simulink library "Contact_Forces_Lib"  (R2025a)
settings: Solver=ode45  StartTime=0.0  StopTime=10.0  RelTol=1e-3  EnableMultiTasking=on
undefined symbols (not defined in the file or in its folder): b_contact, custom_param_1, custom_param_2, Extr_Data_Ring, k_contact, l_cone, length_cylinder, length_tube, mu_kinetic, mu_static, pen_exponent, pen_full_damp_F, rad_s_cone, radius_cylinder, radius_tube, v_thr, X, Y, Z
libraries: nesl_utility x197, sm_lib x115, $bdroot x72, simulink x20, fl_lib x4
(part 3 of 12)

== system Contact_Forces_Lib/2D/Circle to Circle Force Enabled ==
  In : Inport
  Bus Creator : BusCreator  Inputs=7
  Bus Creator1 : BusCreator  Inputs=3
  Bus Selector1 : BusSelector  OutputSignals=Enable
  Calculate Penetration : Subsystem
  External Force and Torque CirB : sm_lib/Forces and Torques/External Force and Torque  EnableForceX=on  EnableForceY=on  EnableForceZ=off  EnableForce=off  ForceResolutionFrame=AttachedFrame  EnableTorqueX=off  EnableTorqueY=off  EnableTorqueZ=on  EnableTorque=off  TorqueResolutionFrame=AttachedFrame
  External Force and Torque CirF : sm_lib/Forces and Torques/External Force and Torque  EnableForceX=on  EnableForceY=on  EnableForceZ=off  EnableForce=off  ForceResolutionFrame=AttachedFrame  EnableTorqueX=off  EnableTorqueY=off  EnableTorqueZ=on  EnableTorque=off  TorqueResolutionFrame=AttachedFrame
  Ff : Subsystem
  Fn : Subsystem
  Force Law : $bdroot/Force Law  SystemSampleTime=-1  LabelModeActiveChoice=Linear  VariantActivationTime=update diagram  EmptyChoice=off  PassThrough=off  PassThroughVariantControl=(default)  EmptyChoiceVariantControl=(default)  AllowFlexibleInterface=on  Latency=0  AutoFrameSizeCalculation=off
  Interval Test : simulink/Logic and Bit Operations/Interval Test  IntervalClosedRight=on  uplimit=active_angle(2)  IntervalClosedLeft=on  lowlimit=active_angle(1)  OutDataTypeStr=uint8
  Product2 : Product  Inputs=3
  Sensing : Subsystem
  Sum : Subsystem
  Sum1 : Sum  Inputs=+-
  Visual CirB : sm_lib/Body Elements/Extruded Solid  ExtrusionType=General  PolygonNumSides=3  PolygonOuterRadius=1  PolygonOuterRadiusUnits=m  ExportEntireGeometry=off  ExtrusionCrossSection=Extr_Data_Ring(cirB_rad,cirB_rad-vis_len_cirBx,active_angle(1),active_angle(2))  ExtrusionCrossSectionUnits=m  ExportConvexHullGeometry=off  ExtrusionLength=vis_len_cirBz  ExtrusionLengthUnits=m  InertiaType=CalculateFromGeometry  BasedOnType=Density  Density=0  DensityUnits=kg/(m^3)  Mass=1  MassUnits=kg  CenterOfMass=[0 0 0]  CenterOfMassUnits=m  MomentsOfInertia=[1 1 1]  MomentsOfInertiaUnits=kg*m^2  ProductsOfInertia=[0 0 0]  ProductsOfInertiaUnits=kg*m^2  GraphicType=FromGeometry  MarkerShape=Sphere  MarkerSize=10  GraphicVisPropType=SimpleVisualProperties  GraphicDiffuseColor=vis_clr  GraphicOpacity=vis_opc*vis_opc_en  GraphicSpecularColor=[0.5 0.5 0.5 1.0]  GraphicAmbientColor=[0.15 0.15 0.15 1.0]  GraphicEmissiveColor=[0.0 0.0 0.0 1.0]  GraphicShininess=75  DoExposeReferenceFrame=on  SerializedFrames=<Frames/>
  Visual CirF : sm_lib/Body Elements/Extruded Solid  ExtrusionType=General  PolygonNumSides=3  PolygonOuterRadius=1  PolygonOuterRadiusUnits=m  ExportEntireGeometry=off  ExtrusionCrossSection=Extr_Data_Ring(cirF_rad,cirF_rad-vis_len_cirFx,0,360)  ExtrusionCrossSectionUnits=m  ExportConvexHullGeometry=off  ExtrusionLength=vis_len_cirFz  ExtrusionLengthUnits=m  InertiaType=CalculateFromGeometry  BasedOnType=Density  Density=0  DensityUnits=kg/(m^3)  Mass=1  MassUnits=kg  CenterOfMass=[0 0 0]  CenterOfMassUnits=m  MomentsOfInertia=[1 1 1]  MomentsOfInertiaUnits=kg*m^2  ProductsOfInertia=[0 0 0]  ProductsOfInertiaUnits=kg*m^2  GraphicType=FromGeometry  MarkerShape=Sphere  MarkerSize=10  GraphicVisPropType=SimpleVisualProperties  GraphicDiffuseColor=vis_clr  GraphicOpacity=vis_opc*vis_opc_en  GraphicSpecularColor=[0.5 0.5 0.5 1.0]  GraphicAmbientColor=[0.15 0.15 0.15 1.0]  GraphicEmissiveColor=[0.0 0.0 0.0 1.0]  GraphicShininess=75  DoExposeReferenceFrame=on  SerializedFrames=<Frames/>
  CirF : PMIOPort  Tag=PMCPort  Side=Left
  CirB : PMIOPort  Tag=PMCPort  Port=2  Side=Right
  Out : Outport  VectorParamsAs1DForOutWhenUnconnected=off
  wires:
  Sensing/6(vazm) -> Ff/7(vazm)
  Sensing/5(wz) -> Ff/6(wz)
  Ff/7(Ff) -> Bus Creator/7  "Friction Force"
  Sensing/4(R) -> Ff/5(R), Fn/2(R)
  Sum1/1 -> Product2/2
  Interval Test/1 -> Product2/3
  Bus Creator1/1 -> Bus Creator/1  "Frame Sep"
  Bus Creator/1 -> Out/1
  Sensing/3(azm) -> Bus Creator1/3, Ff/2(azm), Fn/3(azm), Interval Test/1  "azm"
  Product2/1 -> Ff/1(Fn), Bus Creator/6, Fn/1(Fn)  "Normal Force"
  Calculate Penetration/2(Pen Vel) -> Force Law/2, Bus Creator/3  "Penetration Vel"
  Sensing/2(vrad) -> Calculate Penetration/2(vrad), Bus Creator1/2  "vrad"
  Force Law/2 -> Sum1/2, Bus Creator/4  "Damp Force"
  Sensing/1(rad) -> Ff/4(rad), Calculate Penetration/1(rad), Bus Creator1/1  "rad"
  Force Law/1 -> Bus Creator/5, Sum1/1  "Spr Force"
  Calculate Penetration/1(Pen) -> Ff/3(Pen), Force Law/1, Bus Creator/2  "Penetration"
  Fn/1(FxCirF) -> Sum/1(FnxCirF)
  Fn/2(FyCirF) -> Sum/2(FnyCirF)
  Fn/3(FxCirB) -> Sum/3(FnxCirB)
  Fn/4(FyCirB) -> Sum/4(FnyCirB)
  Ff/1(FxCirF) -> Sum/5(FfxCirF)
  Ff/2(FyCirF) -> Sum/6(FfyCirF)
  Ff/3(FxCirB) -> Sum/7(FfxCirB)
  Ff/4(FyCirB) -> Sum/8(FfyCirB)
  Ff/5(TzCirF) -> Sum/9(TzCirF)
  Ff/6(TzCirB) -> Sum/10(TzCirB)
  In/1 -> Bus Selector1/1
  Bus Selector1/1 -> Product2/1  "<Enable>"
  connections:
  Sensing/LConn1 -- CirF/RConn1 -- Visual CirF/RConn1 -- External Force and Torque CirF/RConn1
  Sensing/LConn2 -- CirB/RConn1 -- Visual CirB/RConn1 -- External Force and Torque CirB/RConn1
  Sum/RConn1 -- External Force and Torque CirF/LConn1
  Sum/RConn2 -- External Force and Torque CirF/LConn2
  Sum/RConn3 -- External Force and Torque CirF/LConn3
  Sum/RConn4 -- External Force and Torque CirB/LConn1
  Sum/RConn5 -- External Force and Torque CirB/LConn2
  Sum/RConn6 -- External Force and Torque CirB/LConn3

== system Contact_Forces_Lib/2D/Circle to Finite Line Force ==
  Bus Creator : BusCreator  Inputs=7
  Bus Creator1 : BusCreator  Inputs=3
  Calculate Penetration : Subsystem
  Demux : Subsystem
  Demux1 : Demux  Outputs=2
  Enable Force : Subsystem
  External Force and Torque Cir : sm_lib/Forces and Torques/External Force and Torque  EnableForceX=on  EnableForceY=on  EnableForceZ=on  EnableForce=off  ForceResolutionFrame=AttachedFrame  EnableTorqueX=off  EnableTorqueY=off  EnableTorqueZ=on  EnableTorque=off  TorqueResolutionFrame=AttachedFrame
  External Force and Torque Lin : sm_lib/Forces and Torques/External Force and Torque  EnableForceX=on  EnableForceY=on  EnableForceZ=on  EnableForce=off  ForceResolutionFrame=AttachedFrame  EnableTorqueX=off  EnableTorqueY=off  EnableTorqueZ=on  EnableTorque=off  TorqueResolutionFrame=AttachedFrame
  Forces : Subsystem
  If : If  NumInputs=2  IfExpression=(u1 > 0 & u2>0)
  Merge : Merge  InitialOutput=0  InputPortOffsets=0
  Merge1 : Merge  InitialOutput=0  InputPortOffsets=0
  No Force : Subsystem
  Sensing : Subsystem
  Transform nX : sm_lib/Frames and Transforms/Rigid Transform  RotationMethod=None  FollAlignAxisA=+X  BaseAlignAxisA=+Y  FollAlignAxisB=+Y  BaseAlignAxisB=+Z  RotationStandardAxis=+Z  RotationAngle=0.0  RotationAngleUnits=deg  RotationArbitraryAxis=[0 0 1]  RotationSequenceAxes=FollowerAxes  RotationSequence=XYX  RotationSequenceAngles=[0 0 0]  RotationSequenceAnglesUnits=deg  RotationMatrix=[1 0 0; 0 1 0; 0 0 1]  Quaternion=[1 0 0 0]  TranslationMethod=StandardAxis  TranslationCartesianOffset=[0 0 0]  TranslationCartesianOffsetUnits=m  TranslationStandardAxis=-X  TranslationStandardOffset=line_depth-vis_len_linBx/2  TranslationStandardOffsetUnits=m  TranslationROffset=0  TranslationROffsetUnits=m  TranslationThetaOffset=0  TranslationThetaOffsetUnits=deg  TranslationZOffset=0  TranslationZOffsetUnits=m
  Transform pX : sm_lib/Frames and Transforms/Rigid Transform  RotationMethod=None  FollAlignAxisA=+X  BaseAlignAxisA=+Y  FollAlignAxisB=+Y  BaseAlignAxisB=+Z  RotationStandardAxis=+Z  RotationAngle=0.0  RotationAngleUnits=deg  RotationArbitraryAxis=[0 0 1]  RotationSequenceAxes=FollowerAxes  RotationSequence=XYX  RotationSequenceAngles=[0 0 0]  RotationSequenceAnglesUnits=deg  RotationMatrix=[1 0 0; 0 1 0; 0 0 1]  Quaternion=[1 0 0 0]  TranslationMethod=StandardAxis  TranslationCartesianOffset=[0 0 0]  TranslationCartesianOffsetUnits=m  TranslationStandardAxis=+X  TranslationStandardOffset=line_depth-vis_len_linBx/2  TranslationStandardOffsetUnits=m  TranslationROffset=0  TranslationROffsetUnits=m  TranslationThetaOffset=0  TranslationThetaOffsetUnits=deg  TranslationZOffset=0  TranslationZOffsetUnits=m
  Visual CirF : sm_lib/Body Elements/Extruded Solid  ExtrusionType=General  PolygonNumSides=3  PolygonOuterRadius=1  PolygonOuterRadiusUnits=m  ExportEntireGeometry=off  ExtrusionCrossSection=Extr_Data_Ring(circle_rad,circle_rad-vis_len_cirFx,0,360)  ExtrusionCrossSectionUnits=m  ExportConvexHullGeometry=off  ExtrusionLength=vis_len_cirFz  ExtrusionLengthUnits=m  InertiaType=CalculateFromGeometry  BasedOnType=Density  Density=0  DensityUnits=kg/(m^3)  Mass=1  MassUnits=kg  CenterOfMass=[0 0 0]  CenterOfMassUnits=m  MomentsOfInertia=[1 1 1]  MomentsOfInertiaUnits=kg*m^2  ProductsOfInertia=[0 0 0]  ProductsOfInertiaUnits=kg*m^2  GraphicType=FromGeometry  MarkerShape=Sphere  MarkerSize=10  GraphicVisPropType=SimpleVisualProperties  GraphicDiffuseColor=vis_clr  GraphicOpacity=vis_opc*vis_opc_en  GraphicSpecularColor=[0.5 0.5 0.5 1.0]  GraphicAmbientColor=[0.15 0.15 0.15 1.0]  GraphicEmissiveColor=[0.0 0.0 0.0 1.0]  GraphicShininess=75  DoExposeReferenceFrame=on  SerializedFrames=<Frames/>
  Visual LinBnX : sm_lib/Body Elements/Brick Solid  BrickDimensions=[vis_len_linBx line_length vis_len_linBz]  BrickDimensionsUnits=m  ExportEntireGeometry=off  InertiaType=CalculateFromGeometry  BasedOnType=Density  Density=0  DensityUnits=kg/(m^3)  Mass=1  MassUnits=kg  CenterOfMass=[0 0 0]  CenterOfMassUnits=m  MomentsOfInertia=[1 1 1]  MomentsOfInertiaUnits=kg*m^2  ProductsOfInertia=[0 0 0]  ProductsOfInertiaUnits=kg*m^2  GraphicType=FromGeometry  MarkerShape=Sphere  MarkerSize=10  GraphicVisPropType=SimpleVisualProperties  GraphicDiffuseColor=vis_clr  GraphicOpacity=vis_opc*vis_opc_en  GraphicSpecularColor=[0.5 0.5 0.5 1.0]  GraphicAmbientColor=[0.15 0.15 0.15 1.0]  GraphicEmissiveColor=[0.0 0.0 0.0 1.0]  GraphicShininess=75  DoExposeReferenceFrame=on  SerializedFrames=<Frames/>
  Visual LinBpX : sm_lib/Body Elements/Brick Solid  BrickDimensions=[vis_len_linBx line_length vis_len_linBz]  BrickDimensionsUnits=m  ExportEntireGeometry=off  InertiaType=CalculateFromGeometry  BasedOnType=Density  Density=0  DensityUnits=kg/(m^3)  Mass=1  MassUnits=kg  CenterOfMass=[0 0 0]  CenterOfMassUnits=m  MomentsOfInertia=[1 1 1]  MomentsOfInertiaUnits=kg*m^2  ProductsOfInertia=[0 0 0]  ProductsOfInertiaUnits=kg*m^2  GraphicType=FromGeometry  MarkerShape=Sphere  MarkerSize=10  GraphicVisPropType=SimpleVisualProperties  GraphicDiffuseColor=vis_clr  GraphicOpacity=vis_opc*vis_opc_en  GraphicSpecularColor=[0.5 0.5 0.5 1.0]  GraphicAmbientColor=[0.15 0.15 0.15 1.0]  GraphicEmissiveColor=[0.0 0.0 0.0 1.0]  GraphicShininess=75  DoExposeReferenceFrame=on  SerializedFrames=<Frames/>
  CirF : PMIOPort  Tag=PMCPort  Side=Left
  LinB : PMIOPort  Tag=PMCPort  Port=2  Side=Right
  Out : Outport  VectorParamsAs1DForOutWhenUnconnected=off
  wires:
  Sensing/6(wz) -> Forces/9(wz)
  Sensing/5(vy) -> Forces/8(vy)
  Forces/2(F) -> Merge/2
  Sensing/4(q) -> Forces/7(Unit Vector)
  Calculate Penetration/3(Pen Vel) -> Bus Creator/2, Forces/5(Vel)  "Penetration Vel"
  Merge/1 -> Demux/1(F)
  If/2 -> No Force/Action
  No Force/2(F) -> Merge/1
  If/1 -> Forces/Action
  Enable Force/1(Enable) -> If/1
  Calculate Penetration/2(Pen) -> Forces/4(Pen), Bus Creator/3, If/2  "Penetration"
  Sensing/1(y) -> Forces/1(M arm), Enable Force/1(y), Bus Creator1/1  "y"
  Calculate Penetration/1(Pos Sign) -> Forces/3(Pos Cmp)
  Calculate Penetration/4(Vel Sign) -> Forces/6(Vel_Cmp)
  Sensing/3(vx) -> Bus Creator1/3, Calculate Penetration/2(vx)  "vx"
  Sensing/2(x) -> Calculate Penetration/1(x), Forces/2(X Sep), Bus Creator1/2  "x"
  Demux/2(FLin) -> Bus Creator/5  "FLin"
  Demux/1(FCir) -> Bus Creator/4  "FCir"
  Bus Creator/1 -> Out/1
  Bus Creator1/1 -> Bus Creator/1  "Frame Sep"
  Demux1/1 -> Bus Creator/6  "Normal Force"
  Demux1/2 -> Bus Creator/7  "Friction Force"
  No Force/1(Fnf) -> Merge1/1
  Forces/1(Fnf) -> Merge1/2
  Merge1/1 -> Demux1/1
  connections:
  External Force and Torque Cir/LConn4 -- Demux/RConn4
  Demux/RConn8 -- External Force and Torque Lin/LConn4
  External Force and Torque Lin/LConn3 -- Demux/RConn7
  Demux/RConn6 -- External Force and Torque Lin/LConn2
  External Force and Torque Lin/LConn1 -- Demux/RConn5
  Demux/RConn3 -- External Force and Torque Cir/LConn3
  External Force and Torque Cir/LConn2 -- Demux/RConn2
  Demux/RConn1 -- External Force and Torque Cir/LConn1
  External Force and Torque Cir/RConn1 -- CirF/RConn1 -- Sensing/LConn1 -- Visual CirF/RConn1
  LinB/RConn1 -- Transform nX/LConn1 -- Transform pX/LConn1 -- External Force and Torque Lin/RConn1 -- Sensing/LConn2
  Transform pX/RConn1 -- Visual LinBpX/RConn1
  Transform nX/RConn1 -- Visual LinBnX/RConn1

== system Contact_Forces_Lib/2D/Circle to Finite Line Force Enabled ==
  In : Inport
  Bus Creator : BusCreator  Inputs=7
  Bus Creator1 : BusCreator  Inputs=3
  Bus Selector1 : BusSelector  OutputSignals=Enable
  Calculate Penetration : Subsystem
  Demux : Subsystem
  Demux1 : Demux  Outputs=2
  Enable Force : Subsystem
  External Force and Torque Cir : sm_lib/Forces and Torques/External Force and Torque  EnableForceX=on  EnableForceY=on  EnableForceZ=on  EnableForce=off  ForceResolutionFrame=AttachedFrame  EnableTorqueX=off  EnableTorqueY=off  EnableTorqueZ=on  EnableTorque=off  TorqueResolutionFrame=AttachedFrame
  External Force and Torque Lin : sm_lib/Forces and Torques/External Force and Torque  EnableForceX=on  EnableForceY=on  EnableForceZ=on  EnableForce=off  ForceResolutionFrame=AttachedFrame  EnableTorqueX=off  EnableTorqueY=off  EnableTorqueZ=on  EnableTorque=off  TorqueResolutionFrame=AttachedFrame
  Forces : Subsystem
  If : If  NumInputs=3  IfExpression=(u1 > 0 & u2>0 & u3>0)
  In1 : InportShadow
  Merge : Merge  InitialOutput=0  InputPortOffsets=0
  Merge1 : Merge  InitialOutput=0  InputPortOffsets=0
  No Force : Subsystem
  Sensing : Subsystem
  Transform nX : sm_lib/Frames and Transforms/Rigid Transform  RotationMethod=None  FollAlignAxisA=+X  BaseAlignAxisA=+Y  FollAlignAxisB=+Y  BaseAlignAxisB=+Z  RotationStandardAxis=+Z  RotationAngle=0.0  RotationAngleUnits=deg  RotationArbitraryAxis=[0 0 1]  RotationSequenceAxes=FollowerAxes  RotationSequence=XYX  RotationSequenceAngles=[0 0 0]  RotationSequenceAnglesUnits=deg  RotationMatrix=[1 0 0; 0 1 0; 0 0 1]  Quaternion=[1 0 0 0]  TranslationMethod=StandardAxis  TranslationCartesianOffset=[0 0 0]  TranslationCartesianOffsetUnits=m  TranslationStandardAxis=-X  TranslationStandardOffset=line_depth-vis_len_linBx/2  TranslationStandardOffsetUnits=m  TranslationROffset=0  TranslationROffsetUnits=m  TranslationThetaOffset=0  TranslationThetaOffsetUnits=deg  TranslationZOffset=0  TranslationZOffsetUnits=m
  Transform pX : sm_lib/Frames and Transforms/Rigid Transform  RotationMethod=None  FollAlignAxisA=+X  BaseAlignAxisA=+Y  FollAlignAxisB=+Y  BaseAlignAxisB=+Z  RotationStandardAxis=+Z  RotationAngle=0.0  RotationAngleUnits=deg  RotationArbitraryAxis=[0 0 1]  RotationSequenceAxes=FollowerAxes  RotationSequence=XYX  RotationSequenceAngles=[0 0 0]  RotationSequenceAnglesUnits=deg  RotationMatrix=[1 0 0; 0 1 0; 0 0 1]  Quaternion=[1 0 0 0]  TranslationMethod=StandardAxis  TranslationCartesianOffset=[0 0 0]  TranslationCartesianOffsetUnits=m  TranslationStandardAxis=+X  TranslationStandardOffset=line_depth-vis_len_linBx/2  TranslationStandardOffsetUnits=m  TranslationROffset=0  TranslationROffsetUnits=m  TranslationThetaOffset=0  TranslationThetaOffsetUnits=deg  TranslationZOffset=0  TranslationZOffsetUnits=m
  Visual CirF : sm_lib/Body Elements/Extruded Solid  ExtrusionType=General  PolygonNumSides=3  PolygonOuterRadius=1  PolygonOuterRadiusUnits=m  ExportEntireGeometry=off  ExtrusionCrossSection=Extr_Data_Ring(circle_rad,circle_rad-vis_len_cirFx,0,360)  ExtrusionCrossSectionUnits=m  ExportConvexHullGeometry=off  ExtrusionLength=vis_len_cirFz  ExtrusionLengthUnits=m  InertiaType=CalculateFromGeometry  BasedOnType=Density  Density=0  DensityUnits=kg/(m^3)  Mass=1  MassUnits=kg  CenterOfMass=[0 0 0]  CenterOfMassUnits=m  MomentsOfInertia=[1 1 1]  MomentsOfInertiaUnits=kg*m^2  ProductsOfInertia=[0 0 0]  ProductsOfInertiaUnits=kg*m^2  GraphicType=FromGeometry  MarkerShape=Sphere  MarkerSize=10  GraphicVisPropType=SimpleVisualProperties  GraphicDiffuseColor=vis_clr  GraphicOpacity=vis_opc*vis_opc_en  GraphicSpecularColor=[0.5 0.5 0.5 1.0]  GraphicAmbientColor=[0.15 0.15 0.15 1.0]  GraphicEmissiveColor=[0.0 0.0 0.0 1.0]  GraphicShininess=75  DoExposeReferenceFrame=on  SerializedFrames=<Frames/>
  Visual LinBnX : sm_lib/Body Elements/Brick Solid  BrickDimensions=[vis_len_linBx line_length vis_len_linBz]  BrickDimensionsUnits=m  ExportEntireGeometry=off  InertiaType=CalculateFromGeometry  BasedOnType=Density  Density=0  DensityUnits=kg/(m^3)  Mass=1  MassUnits=kg  CenterOfMass=[0 0 0]  CenterOfMassUnits=m  MomentsOfInertia=[1 1 1]  MomentsOfInertiaUnits=kg*m^2  ProductsOfInertia=[0 0 0]  ProductsOfInertiaUnits=kg*m^2  GraphicType=FromGeometry  MarkerShape=Sphere  MarkerSize=10  GraphicVisPropType=SimpleVisualProperties  GraphicDiffuseColor=vis_clr  GraphicOpacity=vis_opc*vis_opc_en  GraphicSpecularColor=[0.5 0.5 0.5 1.0]  GraphicAmbientColor=[0.15 0.15 0.15 1.0]  GraphicEmissiveColor=[0.0 0.0 0.0 1.0]  GraphicShininess=75  DoExposeReferenceFrame=on  SerializedFrames=<Frames/>
  Visual LinBpX : sm_lib/Body Elements/Brick Solid  BrickDimensions=[vis_len_linBx line_length vis_len_linBz]  BrickDimensionsUnits=m  ExportEntireGeometry=off  InertiaType=CalculateFromGeometry  BasedOnType=Density  Density=0  DensityUnits=kg/(m^3)  Mass=1  MassUnits=kg  CenterOfMass=[0 0 0]  CenterOfMassUnits=m  MomentsOfInertia=[1 1 1]  MomentsOfInertiaUnits=kg*m^2  ProductsOfInertia=[0 0 0]  ProductsOfInertiaUnits=kg*m^2  GraphicType=FromGeometry  MarkerShape=Sphere  MarkerSize=10  GraphicVisPropType=SimpleVisualProperties  GraphicDiffuseColor=vis_clr  GraphicOpacity=vis_opc*vis_opc_en  GraphicSpecularColor=[0.5 0.5 0.5 1.0]  GraphicAmbientColor=[0.15 0.15 0.15 1.0]  GraphicEmissiveColor=[0.0 0.0 0.0 1.0]  GraphicShininess=75  DoExposeReferenceFrame=on  SerializedFrames=<Frames/>
  CirF : PMIOPort  Tag=PMCPort  Side=Left
  LinB : PMIOPort  Tag=PMCPort  Port=2  Side=Right
  Out : Outport  VectorParamsAs1DForOutWhenUnconnected=off
  wires:
  Merge1/1 -> Demux1/1
  Forces/1(Fnf) -> Merge1/2
  No Force/1(Fnf) -> Merge1/1
  Demux1/2 -> Bus Creator/7  "Friction Force"
  Demux1/1 -> Bus Creator/6  "Normal Force"
  Bus Creator1/1 -> Bus Creator/1  "Frame Sep"
  Bus Creator/1 -> Out/1
  Demux/1(FCir) -> Bus Creator/4  "FCir"
  Demux/2(FLin) -> Bus Creator/5  "FLin"
  Sensing/2(x) -> Bus Creator1/2, Forces/2(X Sep), Calculate Penetration/1(x)  "x"
  Sensing/3(vx) -> Calculate Penetration/2(vx), Bus Creator1/3  "vx"
  Calculate Penetration/4(Vel Sign) -> Forces/6(Vel_Cmp)
  Calculate Penetration/1(Pos Sign) -> Forces/3(Pos Cmp)
  Sensing/1(y) -> Bus Creator1/1, Enable Force/1(y), Forces/1(M arm)  "y"
  Calculate Penetration/2(Pen) -> If/3, Bus Creator/3, Forces/4(Pen)  "Penetration"
  Enable Force/1(Enable) -> If/2
  If/1 -> Forces/Action
  No Force/2(F) -> Merge/1
  If/2 -> No Force/Action
  Merge/1 -> Demux/1(F)
  Calculate Penetration/3(Pen Vel) -> Forces/5(Vel), Bus Creator/2  "Penetration Vel"
  Sensing/4(q) -> Forces/7(Unit Vector)
  Forces/2(F) -> Merge/2
  Sensing/5(vy) -> Forces/8(vy)
  Sensing/6(wz) -> Forces/9(wz)
  Bus Selector1/1 -> If/1  "<Enable>"
  In/1 -> Bus Selector1/1
  In1/1 -> Sensing/1(In)
  connections:
  Transform nX/RConn1 -- Visual LinBnX/RConn1
  Transform pX/RConn1 -- Visual LinBpX/RConn1
  Sensing/LConn2 -- External Force and Torque Lin/RConn1 -- Transform pX/LConn1 -- Transform nX/LConn1 -- LinB/RConn1
  Visual CirF/RConn1 -- CirF/RConn1 -- Sensing/LConn1 -- External Force and Torque Cir/RConn1
  Demux/RConn1 -- External Force and Torque Cir/LConn1
  External Force and Torque Cir/LConn2 -- Demux/RConn2
  Demux/RConn3 -- External Force and Torque Cir/LConn3
  External Force and Torque Lin/LConn1 -- Demux/RConn5
  Demux/RConn6 -- External Force and Torque Lin/LConn2
  External Force and Torque Lin/LConn3 -- Demux/RConn7
  Demux/RConn8 -- External Force and Torque Lin/LConn4
  External Force and Torque Cir/LConn4 -- Demux/RConn4

== system Contact_Forces_Lib/2D/Circle to Hole Force ==
  Attraction Force : $bdroot/Other Forces/Attraction Force  k_pen=k_contact  b_penvel=b_contact  max_sep=max_frame_sep  deadzone=h_deadzone
  Bus Creator : BusCreator  Inputs=6
  Bus Creator1 : BusCreator  Inputs=3
  Calculate Penetration : Subsystem
  Internal Force : sm_lib/Forces and Torques/Internal Force
  Interval Test : simulink/Logic and Bit Operations/Interval Test  IntervalClosedRight=on  uplimit=active_angle(2)  IntervalClosedLeft=on  lowlimit=active_angle(1)  OutDataTypeStr=uint8
  Product : Product
  Sensing : Subsystem
  Simulink-PS Converter2 : nesl_utility/Simulink-PS Converter  PhysicalDomain=network_engine_domain  SubClassName=ps_input  LeftPortType=input  RightPortType=output  PseudoPeriodic=off  Frequencies=[]  NoiseDistribution=none  NoiseParameters=[]  Unit=1  AffineConversion=off  FilteringAndDerivatives=zero  SimscapeFilterOrder=1  InputFilterTimeConstant=0.005  UdotUserProvided=[]
  Sum : Sum  Inputs=+-
  Terminator : Terminator
  CirF : PMIOPort  Tag=PMCPort  Side=Left
  CirB : PMIOPort  Tag=PMCPort  Port=2  Side=Right
  Out : Outport  VectorParamsAs1DForOutWhenUnconnected=off
  wires:
  Interval Test/1 -> Product/2
  Sensing/3(q) -> Terminator/1
  Sum/1 -> Product/1
  Attraction Force/1 -> Bus Creator/5, Sum/1  "Spr Force"
  Sensing/1(rad) -> Bus Creator1/1, Calculate Penetration/1(Pos)  "rad"
  Attraction Force/2 -> Bus Creator/4, Sum/2  "Damp Force"
  Sensing/2(vrad) -> Bus Creator1/2, Calculate Penetration/2(Vel)  "vrad"
  Calculate Penetration/2(Pen Vel) -> Attraction Force/2, Bus Creator/3  "Penetration Vel"
  Product/1 -> Bus Creator/6, Simulink-PS Converter2/1  "Total Force"
  Sensing/4(azm) -> Bus Creator1/3, Interval Test/1  "azm"
  Bus Creator1/1 -> Bus Creator/1  "Frame Sep"
  Calculate Penetration/1(Pen) -> Attraction Force/1, Bus Creator/2  "Penetration"
  Bus Creator/1 -> Out/1
  connections:
  Sensing/LConn2 -- Internal Force/RConn1 -- CirB/RConn1
  Internal Force/LConn1 -- Sensing/LConn1 -- CirF/RConn1
  Simulink-PS Converter2/RConn1 -- Internal Force/LConn2

== system Contact_Forces_Lib/2D/Circle to Ring Force ==
  Bus Creator1 : BusCreator  Inputs=3
  Check Active : Subsystem
  Check Active Range : Subsystem
  External Force and Torque CirF : sm_lib/Forces and Torques/External Force and Torque  EnableForceX=on  EnableForceY=on  EnableForceZ=off  EnableForce=off  ForceResolutionFrame=AttachedFrame  EnableTorqueX=off  EnableTorqueY=off  EnableTorqueZ=on  EnableTorque=off  TorqueResolutionFrame=AttachedFrame
  External Force and Torque RinB : sm_lib/Forces and Torques/External Force and Torque  EnableForceX=on  EnableForceY=on  EnableForceZ=off  EnableForce=off  ForceResolutionFrame=AttachedFrame  EnableTorqueX=off  EnableTorqueY=off  EnableTorqueZ=on  EnableTorque=off  TorqueResolutionFrame=AttachedFrame
  Forces : Subsystem
  If : If  IfExpression=u1
  Merge : Merge  InitialOutput=0  InputPortOffsets=0
  No Force : Subsystem
  Sensing : Subsystem
  Subsystem : Subsystem
  Visual CirF Outer : sm_lib/Body Elements/Extruded Solid  ExtrusionType=General  PolygonNumSides=3  PolygonOuterRadius=1  PolygonOuterRadiusUnits=m  ExportEntireGeometry=off  ExtrusionCrossSection=Extr_Data_Ring(radius_circle,radius_circle-vis_len_cirFx,0,360)  ExtrusionCrossSectionUnits=m  ExportConvexHullGeometry=off  ExtrusionLength=vis_len_cirFz  ExtrusionLengthUnits=m  InertiaType=CalculateFromGeometry  BasedOnType=Density  Density=0  DensityUnits=kg/(m^3)  Mass=1  MassUnits=kg  CenterOfMass=[0 0 0]  CenterOfMassUnits=m  MomentsOfInertia=[1 1 1]  MomentsOfInertiaUnits=kg*m^2  ProductsOfInertia=[0 0 0]  ProductsOfInertiaUnits=kg*m^2  GraphicType=FromGeometry  MarkerShape=Sphere  MarkerSize=10  GraphicVisPropType=SimpleVisualProperties  GraphicDiffuseColor=vis_clr  GraphicOpacity=vis_opc*vis_opc_en  GraphicSpecularColor=[0.5 0.5 0.5 1.0]  GraphicAmbientColor=[0.15 0.15 0.15 1.0]  GraphicEmissiveColor=[0.0 0.0 0.0 1.0]  GraphicShininess=75  DoExposeReferenceFrame=on  SerializedFrames=<Frames/>
  Visual RinB Inner : sm_lib/Body Elements/Extruded Solid  ExtrusionType=General  PolygonNumSides=3  PolygonOuterRadius=1  PolygonOuterRadiusUnits=m  ExportEntireGeometry=off  ExtrusionCrossSection=Extr_Data_Ring(radius_ring-d_ring/2+vis_len_rinBx,radius_ring-d_ring/2,active_angle(1),active_angle(2))  ExtrusionCrossSectionUnits=m  ExportConvexHullGeometry=off  ExtrusionLength=vis_len_rinBz  ExtrusionLengthUnits=m  InertiaType=CalculateFromGeometry  BasedOnType=Density  Density=0  DensityUnits=kg/(m^3)  Mass=1  MassUnits=kg  CenterOfMass=[0 0 0]  CenterOfMassUnits=m  MomentsOfInertia=[1 1 1]  MomentsOfInertiaUnits=kg*m^2  ProductsOfInertia=[0 0 0]  ProductsOfInertiaUnits=kg*m^2  GraphicType=FromGeometry  MarkerShape=Sphere  MarkerSize=10  GraphicVisPropType=SimpleVisualProperties  GraphicDiffuseColor=vis_clr  GraphicOpacity=vis_opc*vis_opc_en  GraphicSpecularColor=[0.5 0.5 0.5 1.0]  GraphicAmbientColor=[0.15 0.15 0.15 1.0]  GraphicEmissiveColor=[0.0 0.0 0.0 1.0]  GraphicShininess=75  DoExposeReferenceFrame=on  SerializedFrames=<Frames/>
  Visual RinB Outer : sm_lib/Body Elements/Extruded Solid  ExtrusionType=General  PolygonNumSides=3  PolygonOuterRadius=1  PolygonOuterRadiusUnits=m  ExportEntireGeometry=off  ExtrusionCrossSection=Extr_Data_Ring(radius_ring+d_ring/2,radius_ring+d_ring/2-vis_len_rinBx,active_angle(1),active_angle(2))  ExtrusionCrossSectionUnits=m  ExportConvexHullGeometry=off  ExtrusionLength=vis_len_rinBz  ExtrusionLengthUnits=m  InertiaType=CalculateFromGeometry  BasedOnType=Density  Density=0  DensityUnits=kg/(m^3)  Mass=1  MassUnits=kg  CenterOfMass=[0 0 0]  CenterOfMassUnits=m  MomentsOfInertia=[1 1 1]  MomentsOfInertiaUnits=kg*m^2  ProductsOfInertia=[0 0 0]  ProductsOfInertiaUnits=kg*m^2  GraphicType=FromGeometry  MarkerShape=Sphere  MarkerSize=10  GraphicVisPropType=SimpleVisualProperties  GraphicDiffuseColor=vis_clr  GraphicOpacity=vis_opc*vis_opc_en  GraphicSpecularColor=[0.5 0.5 0.5 1.0]  GraphicAmbientColor=[0.15 0.15 0.15 1.0]  GraphicEmissiveColor=[0.0 0.0 0.0 1.0]  GraphicShininess=75  DoExposeReferenceFrame=on  SerializedFrames=<Frames/>
  CirF : PMIOPort  Tag=PMCPort  Side=Left
  RinB : PMIOPort  Tag=PMCPort  Port=2  Side=Right
  Out : Outport  VectorParamsAs1DForOutWhenUnconnected=off
  wires:
  Check Active/1(Out) -> Out/1
  Bus Creator1/1 -> Check Active/3(PosVel)  "Frame Sep"
  Forces/2(Out) -> Check Active/1(Force)
  Sensing/4(vazm) -> Forces/4(vazm)
  Sensing/1(rad) -> Bus Creator1/1, Forces/1(rad)  "rad"
  Sensing/6(R) -> Forces/6(R)
  Forces/1(Frc) -> Merge/2
  No Force/1(F) -> Merge/1
  Check Active Range/1(En) -> If/1, Check Active/2(Active)
  If/1 -> Forces/Action
  If/2 -> No Force/Action
  Sensing/3(azm) -> Bus Creator1/3, Check Active Range/1(azm), Forces/3(azm)  "azm"
  Sensing/2(vrad) -> Bus Creator1/2, Forces/2(vrad)  "vrad"
  Sensing/5(wzf) -> Forces/5(wzf)
  Merge/1 -> Subsystem/1(Frc)  "Total Force"
  connections:
  Subsystem/RConn2 -- External Force and Torque CirF/LConn2
  Subsystem/RConn3 -- External Force and Torque CirF/LConn3
  Subsystem/RConn6 -- External Force and Torque RinB/LConn3
  Subsystem/RConn1 -- External Force and Torque CirF/LConn1
  Subsystem/RConn4 -- External Force and Torque RinB/LConn1
  Subsystem/RConn5 -- External Force and Torque RinB/LConn2
  Sensing/LConn2 -- External Force and Torque RinB/RConn1 -- Visual RinB Outer/RConn1 -- Visual RinB Inner/RConn1 -- RinB/RConn1
  Sensing/LConn1 -- External Force and Torque CirF/RConn1 -- Visual CirF Outer/RConn1 -- CirF/RConn1

== system Contact_Forces_Lib/2D/Composite Forces ==
  Box to Belt Force : Subsystem  mask(Box to Belt Contact Force){box_l=0.3, box_h=0.1, belt_l=3, belt_h=0.2, contact_circle_rad_box2belt=0, force_law_box2belt=Linear, k_contact_box2belt=1e4, b_contact_box2belt=1e2, pen_full_damp_F_box2belt=1e-4, pen_exponent_box2belt=1, friction_law_box2belt=Stick-Slip Continuous, mu_kinetic_box2belt=0.35, mu_static_box2belt=0.4, v_thr_box2belt=0.001, vis_on_box2belt=off, vis_opc_en_box2belt=0, vis_len_boxz=0.1, vis_len_boxx=0.005, vis_len_beltz=0.1, vis_len_beltx=0.005, vis_clr_box2belt=[0.9 0.2 0.2], vis_opc_box2belt=0.7}
      mask prompts: box_l "Box Length (m)"; box_h "Box Height (m)"; belt_l "Belt Length (m)"; belt_h "Belt Height (m)"; contact_circle_rad_box2belt "Box Contact Circle Radius (m)"; force_law_box2belt "Force Law"; k_contact_box2belt "Contact Stiffness (N/m)"; b_contact_box2belt "Contact Damping (N/(m/s))"; pen_full_damp_F_box2belt "Penetration for full damping (m)"; pen_exponent_box2belt "Penetration exponent (>=1)"; friction_law_box2belt "Friction Law"; mu_kinetic_box2belt "Coefficient of Kinetic Friction"; mu_static_box2belt "Coefficient of Static Friction"; v_thr_box2belt "Velocity Threshold (m/s)"; vis_on_box2belt "Visualize Contact Surfaces"; vis_opc_en_box2belt "Visualize Opacity Enable"; vis_clr_box2belt "Color of Surface Element (RGB)"; vis_opc_box2belt "Opacity of Surface Element (0-1)"
      mask help:
      | This subsystem models planar contact forces between a box and a conveyor belt.  The conveyor belt moves at the speed specified by the input signal in m/s.
      |
      | Click the Help button for a diagram of the contact forces and the parameters.
      mask init:
      | contact_circle_rad_box2belt=min([box_l box_h])*0.05;
      | 
      | f=Simulink.FindOptions('FollowLinks',0,'LookUnderMasks','all','RegExp',1);
      | CR_bpth=Simulink.findBlocks(gcb,'friction_law','.*',f);
      | 
      | if(~isempty(CR_bpth))
      |     temp_frlaw = get_param(gcb,'friction_law_box2belt');
      |     for i=1:length(CR_bpth)
      |         set_param(CR_bpth(i),'friction_law',temp_frlaw);
      |     end
      |     clear temp_frlaw
      | 
      |     temp_forcelaw = get_param(gcb,'force_law_box2belt');
      |     for i=1:length(CR_bpth)
      |         set_param(CR_bpth(i),'force_law',temp_forcelaw);
      |     end
      |     clear temp_forcelaw
      | 
      |     temp_vis_on = get_param(gcb,'vis_on_box2belt');
      |     for i=1:length(CR_bpth)
      |         set_param(CR_bpth(i),'vis_on',temp_vis_on);
      |     end
      |     clear temp_vis_on
      | end
      mask Help: web(which('Box_to_Belt_Contact.html'));
      mask TypeOptions force_law_box2belt: Linear | Nonlinear
      mask Callback force_law_box2belt:
      | maskObj = Simulink.Mask.get(gcb);
      | pfd_h = maskObj.getParameter('pen_full_damp_F_box2belt');
      | pex_h = maskObj.getParameter('pen_exponent_box2belt');
      | if strcmp(get_param(gcb,'force_law_box2belt'),'Linear')
      |     pfd_h.Visible = 'off';
      |     pex_h.Visible = 'off';
      | elseif strcmp(get_param(gcb,'force_law_box2belt'),'Nonlinear')
      |     pfd_h.Visible = 'on';
      |     pex_h.Visible = 'on';
      | end
      mask TypeOptions friction_law_box2belt: None | Stick-Slip Continuous
      mask Callback friction_law_box2belt:
      | maskObj = Simulink.Mask.get(gcb);
      | muk_h = maskObj.getParameter('mu_kinetic_box2belt');
      | mus_h = maskObj.getParameter('mu_static_box2belt');
      | vth_h = maskObj.getParameter('v_thr_box2belt');
      | if strcmp(get_param(gcb,'friction_law_box2belt'),'None')
      |     muk_h.Visible = 'off';
      |     mus_h.Visible = 'off';
      |     vth_h.Visible = 'off';
      | elseif strcmp(get_param(gcb,'friction_law_box2belt'),'Stick-Slip Continuous')
      |     muk_h.Visible = 'on';
      |     mus_h.Visible = 'on';
      |     vth_h.Visible = 'on';
      | end
      | clear maskObj
      mask Callback vis_on_box2belt:
      | maskObj = Simulink.Mask.get(gcb);
      | 
      | vis_len_prompt_h = maskObj.getDialogControl('vis_len_prompt_box2belt');
      | vis_len_promptZaxis_h = maskObj.getDialogControl('vis_len_promptZaxis');
      | vis_len_promptXaxis_h = maskObj.getDialogControl('vis_len_promptXaxis');
      | vis_len_promptBox_h = maskObj.getDialogControl('vis_len_promptBox');
      | vis_len_promptBelt_h = maskObj.getDialogControl('vis_len_promptBelt');
      | vis_len_boxz_h = maskObj.getParameter('vis_len_boxz');
      | vis_len_boxx_h = maskObj.getParameter('vis_len_boxx');
      | vis_len_beltz_h = maskObj.getParameter('vis_len_beltz');
      | vis_len_beltx_h = maskObj.getParameter('vis_len_beltx');
      | vis_clr_box2belt_h = maskObj.getParameter('vis_clr_box2belt');
      | vis_opc_box2belt_h = maskObj.getParameter('vis_opc_box2belt');
      | 
      | temp_visCBstate = get_param(gcb,'vis_on_box2belt');
      | vis_len_prompt_h.Visible = temp_visCBstate;
      | vis_len_promptZaxis_h.Visible = temp_visCBstate;
      | vis_len_promptXaxis_h.Visible = temp_visCBstate;
      | vis_len_promptBox_h.Visible = temp_visCBstate;
      | vis_len_promptBelt_h.Visible = temp_visCBstate;
      | vis_len_boxz_h.Visible = temp_visCBstate;
      | vis_len_boxx_h.Visible = temp_visCBstate;
      | vis_len_beltz_h.Visible = temp_visCBstate;
      | vis_len_beltx_h.Visible = temp_visCBstate;
      | vis_clr_box2belt_h.Visible = temp_visCBstate;
      | vis_opc_box2belt_h.Visible = temp_visCBstate;
      | 
      | clear maskObj vis_clr_box2belt_h vis_opc_box2belt_h
      | clear vis_len_prompt_h temp_visCBstate
      | clear vis_len_promptZaxis_h vis_len_promptXaxis_h
      | clear vis_len_promptBox_h vis_len_promptBelt_h
      | clear vis_len_boxz_h vis_len_boxx_h
      | clear vis_len_beltz_h vis_len_beltx_h
      mask DialogControl Container4 Prompt: Dimensions
      mask DialogControl Container5 Prompt: Contact
      mask DialogControl frict_container Prompt: Friction
      mask DialogControl Vis_Cont Prompt: Visual
      mask DialogControl vis_len_prompt_box2belt Prompt: Length of Surface
      mask DialogControl vis_len_promptZaxis Prompt: Z-Axis (m)
      mask DialogControl vis_len_promptXaxis Prompt: X-Axis (m)
      mask DialogControl vis_len_promptBox Prompt: Box
      mask DialogControl vis_len_promptBelt Prompt: Belt
      mask Display: image('Box_to_Belt_Contact_IMAGE.jpg');
  Box to Box Force : Subsystem  mask(Box to Box Contact Force){boxB_l=0.3, boxB_h=0.3, boxF_l=0.2, boxF_h=0.1, boxB_contact_rad=0, boxF_contact_rad=0, force_law_box2box=Linear, k_contact_box2box=1e4, b_contact_box2box=1e2, pen_full_damp_F_box2box=1e-4, pen_exponent_box2box=1, friction_law_box2box=None, mu_kinetic_box2box=0.5, mu_static_box2box=0.7, v_thr_box2box=0.001, vis_on_box2box=off, vis_opc_en_box2box=0, vis_len_boxBz=0.1, vis_len_boxBx=0.005, vis_len_boxFz=0.1, vis_len_boxFx=0.005, vis_clr_box2box=[0.9 0.2 0.2], vis_opc_box2box=0.7}
      mask prompts: boxB_l "BoxB length x (m)"; boxB_h "BoxB length y (m)"; boxF_l "BoxF length x (m)"; boxF_h "BoxF length y (m)"; boxB_contact_rad "Base Box Contact Circle Radius (m)"; boxF_contact_rad "Follower Box Contact Circle Radius (m)"; force_law_box2box "Force Law"; k_contact_box2box "Contact Stiffness (N/m)"; b_contact_box2box "Contact Damping (N/(m/s))"; pen_full_damp_F_box2box "Penetration for full damping (m)"; pen_exponent_box2box "Penetration exponent (>=1)"; friction_law_box2box "Friction Law"; mu_kinetic_box2box "Coefficient of Kinetic Friction"; mu_static_box2box "Coefficient of Static Friction"; v_thr_box2box "Velocity Threshold (m/s)"; vis_on_box2box "Visualize Contact Surfaces"; vis_opc_en_box2box "Visualize Opacity Enable"; vis_clr_box2box "Color of Surface Element (RGB)"; vis_opc_box2box "Opacity of Surface Element (0-1)"
      mask help:
      | This subsystem models planar contact forces between two boxes.
      |
      | Click the Help button for a diagram of the contact forces and the parameters.
      mask init:
      | boxB_contact_rad=min([boxB_h boxB_l])*0.05;
      | boxF_contact_rad=min([boxF_h boxF_l])*0.05;
      | 
      | f=Simulink.FindOptions('FollowLinks',0,'LookUnderMasks','all','RegExp',1);
      | CR_bpth=Simulink.findBlocks(gcb,'friction_law','.*',f);
      | 
      | if(~isempty(CR_bpth))
      |     temp_frlaw = get_param(gcb,'friction_law_box2box');
      |     for i=1:length(CR_bpth)
      |         set_param(CR_bpth(i),'friction_law',temp_frlaw);
      |     end
      |     clear temp_frlaw
      | 
      |     temp_forcelaw = get_param(gcb,'force_law_box2box');
      |     for i=1:length(CR_bpth)
      |         set_param(CR_bpth(i),'force_law',temp_forcelaw);
      |     end
      |     clear temp_forcelaw
      | 
      |     temp_vis_on = get_param(gcb,'vis_on_box2box');
      |     for i=1:length(CR_bpth)
      |         set_param(CR_bpth(i),'vis_on',temp_vis_on);
      |     end
      |     clear temp_vis_on
      | end
      mask Help: web(which('Box_to_Box_Contact.html'));
      mask TypeOptions force_law_box2box: Linear | Nonlinear
      mask Callback force_law_box2box:
      | maskObj = Simulink.Mask.get(gcb);
      | pfd_h = maskObj.getParameter('pen_full_damp_F_box2box');
      | pex_h = maskObj.getParameter('pen_exponent_box2box');
      | if strcmp(get_param(gcb,'force_law_box2box'),'Linear')
      |     pfd_h.Visible = 'off';
      |     pex_h.Visible = 'off';
      | elseif strcmp(get_param(gcb,'force_law_box2box'),'Nonlinear')
      |     pfd_h.Visible = 'on';
      |     pex_h.Visible = 'on';
      | end
      mask TypeOptions friction_law_box2box: None | Stick-Slip Continuous
      mask Callback friction_law_box2box:
      | maskObj = Simulink.Mask.get(gcb);
      | muk_h = maskObj.getParameter('mu_kinetic_box2box');
      | mus_h = maskObj.getParameter('mu_static_box2box');
      | vth_h = maskObj.getParameter('v_thr_box2box');
      | if strcmp(get_param(gcb,'friction_law_box2box'),'None')
      |     muk_h.Visible = 'off';
      |     mus_h.Visible = 'off';
      |     vth_h.Visible = 'off';
      | elseif strcmp(get_param(gcb,'friction_law_box2box'),'Stick-Slip Continuous')
      |     muk_h.Visible = 'on';
      |     mus_h.Visible = 'on';
      |     vth_h.Visible = 'on';
      | end
      | clear maskObj
      mask Callback vis_on_box2box:
      | maskObj = Simulink.Mask.get(gcb);
      | 
      | vis_len_prompt_h = maskObj.getDialogControl('vis_len_prompt_box2box');
      | vis_len_promptZaxis_h = maskObj.getDialogControl('vis_len_promptZaxis');
      | vis_len_promptXaxis_h = maskObj.getDialogControl('vis_len_promptXaxis');
      | vis_len_promptBase_h = maskObj.getDialogControl('vis_len_promptBase');
      | vis_len_promptFollower_h = maskObj.getDialogControl('vis_len_promptFollower');
      | vis_len_boxBz_h = maskObj.getParameter('vis_len_boxBz');
      | vis_len_boxBx_h = maskObj.getParameter('vis_len_boxBx');
      | vis_len_boxFz_h = maskObj.getParameter('vis_len_boxFz');
      | vis_len_boxFx_h = maskObj.getParameter('vis_len_boxFx');
      | vis_clr_box2box_h = maskObj.getParameter('vis_clr_box2box');
      | vis_opc_box2box_h = maskObj.getParameter('vis_opc_box2box');
      | 
      | temp_visCBstate = get_param(gcb,'vis_on_box2box');
      | vis_len_prompt_h.Visible = temp_visCBstate;
      | vis_len_promptZaxis_h.Visible = temp_visCBstate;
      | vis_len_promptXaxis_h.Visible = temp_visCBstate;
      | vis_len_promptBase_h.Visible = temp_visCBstate;
      | vis_len_promptFollower_h.Visible = temp_visCBstate;
      | vis_len_boxBz_h.Visible = temp_visCBstate;
      | vis_len_boxBx_h.Visible = temp_visCBstate;
      | vis_len_boxFz_h.Visible = temp_visCBstate;
      | vis_len_boxFx_h.Visible = temp_visCBstate;
      | vis_clr_box2box_h.Visible = temp_visCBstate;
      | vis_opc_box2box_h.Visible = temp_visCBstate;
      | 
      | clear maskObj vis_clr_box2box_h vis_opc_box2box_h
      | clear vis_len_prompt_h temp_visCBstate
      | clear vis_len_promptZaxis_h vis_len_promptXaxis_h
      | clear vis_len_promptBase_h vis_len_promptFollower_h
      | clear vis_len_boxBz_h vis_len_boxBx_h
      | clear vis_len_boxFz_h vis_len_boxFx_h
      mask DialogControl Container4 Prompt: Dimensions
      mask DialogControl Container6 Prompt: Contact
      mask DialogControl Container7 Prompt: Friction
      mask DialogControl Vis_Cont Prompt: Visual
      mask DialogControl vis_len_prompt_box2box Prompt: Length of Surface
      mask DialogControl vis_len_promptZaxis Prompt: Z-Axis (m)
      mask DialogControl vis_len_promptXaxis Prompt: X-Axis (m)
      mask DialogControl vis_len_promptBase Prompt: Base
      mask DialogControl vis_len_promptFollower Prompt: Follower
      mask Display: image('Box_to_Box_Contact_IMAGE.jpg');
